simulink model "cable_driven_parallel_robot"  (R2023a)
settings: Solver=ode3  StartTime=0.0  StopTime=100  FixedStep=0.01  RelTol=1e-3
values from neighbouring files (symbols this model uses):
  cable_length = 1.2    [Model_Info.m]
  g = 9.81    [Model_Info.m]
  MP_H = 2    [Model_Info.m]
  MP_init_X = 0    [Model_Info.m]
  MP_init_Y = 0    [Model_Info.m]
  MP_init_Z = cable_length + (MP_H/2)    (= 2.2)    [Model_Info.m]
  MP_Ix = (MP_m/12)*(MP_W^2+MP_H^2)    (= 6.66666666667e-05)    [Model_Info.m]
  MP_Iy = (MP_m/12)*(MP_L^2+MP_H^2)    (= 6.66666666667e-05)    [Model_Info.m]
  MP_Iz = (MP_m/12)*(MP_L^2+MP_W^2)    (= 6.66666666667e-05)    [Model_Info.m]
  MP_L = 2    [Model_Info.m]
  MP_m = 0.0001    [Model_Info.m]
  MP_W = 2    [Model_Info.m]
  MR_init_X_L1 = -(MP_L/2)    (= -1)    [Model_Info.m]
  MR_init_X_L2 = (MP_L/2)    (= 1)    [Model_Info.m]
  MR_init_X_L3 = (MP_L/2)    (= 1)    [Model_Info.m]
  MR_init_X_L4 = -(MP_L/2)    (= -1)    [Model_Info.m]
  MR_init_Y_L1 = -(MP_W/2)    (= -1)    [Model_Info.m]
  MR_init_Y_L2 = -(MP_W/2)    (= -1)    [Model_Info.m]
  MR_init_Y_L3 = (MP_W/2)    (= 1)    [Model_Info.m]
  MR_init_Y_L4 = (MP_W/2)    (= 1)    [Model_Info.m]
  MR_init_Yaw_L1 = pi    (= 3.14159265359)    [Model_Info.m]
  MR_init_Yaw_L2 = 0    [Model_Info.m]
  MR_init_Yaw_L3 = 0    [Model_Info.m]
  MR_init_Yaw_L4 = pi    (= 3.14159265359)    [Model_Info.m]
  MR_Jr = (MR_m/12)*(MR_L^2+MR_W^2)    (= 0.333333333333)    [Model_Info.m]
  MR_m = 0.5    [Model_Info.m]
  MR_r = 2    [Model_Info.m]
  MR_WT = 2    [Model_Info.m]
  QR_Ax = 0.25*0    (= 0)    [Model_Info.m]
  QR_Ay = 0.25*0    (= 0)    [Model_Info.m]
  QR_Az = 0.25*0    (= 0)    [Model_Info.m]
  QR_b = 1.14*1e-7    (= 1.14e-07)    [Model_Info.m]
  QR_Ixx = 4.856*1e-3    (= 0.004856)    [Model_Info.m]
  QR_Iyy = 4.856*1e-3    (= 0.004856)    [Model_Info.m]
  QR_Izz = 8.801*1e-3    (= 0.008801)    [Model_Info.m]
  QR_K = 2.980*1e-6    (= 2.98e-06)    [Model_Info.m]
  QR_l = 0.225    [Model_Info.m]
  QR_m = 0.468    [Model_Info.m]
  QR_x0_U1 = -(MP_L/2)    (= -1)    [Model_Info.m]
  QR_x0_U2 = (MP_L/2)    (= 1)    [Model_Info.m]
  QR_x0_U3 = (MP_L/2)    (= 1)    [Model_Info.m]
  QR_x0_U4 = -(MP_L/2)    (= -1)    [Model_Info.m]
  QR_y0_U1 = -(MP_W/2)    (= -1)    [Model_Info.m]
  QR_y0_U2 = -(MP_W/2)    (= -1)    [Model_Info.m]
  QR_y0_U3 = (MP_W/2)    (= 1)    [Model_Info.m]
  QR_y0_U4 = (MP_W/2)    (= 1)    [Model_Info.m]
  QR_z0_U1 = 2*cable_length+(MP_H)    (= 4.4)    [Model_Info.m]
  QR_z0_U2 = 2*cable_length+(MP_H)    (= 4.4)    [Model_Info.m]
  QR_z0_U3 = 2*cable_length+(MP_H)    (= 4.4)    [Model_Info.m]
  QR_z0_U4 = 2*cable_length+(MP_H)    (= 4.4)    [Model_Info.m]
(part 1 of 12)
settings Model: Creator=ahmed  LastModifiedBy=Siddharth U
settings SolverCC: AlgebraicLoopSolver=TrustRegion
settings DebuggingCC: UnconnectedInputMsg=warning  UnconnectedOutputMsg=warning  UnconnectedLineMsg=warning  UnderSpecifiedDimensionMsg=warning
settings ModelReferenceCC: EnableRefExpFcnMdlSchedulingChecks=on

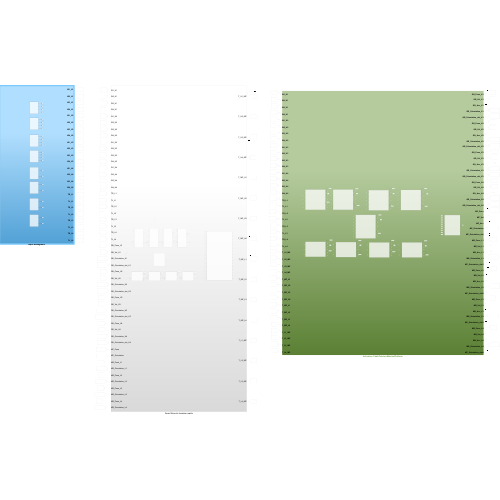
[thumbnail: Simulink's stored preview of the top-level diagram]
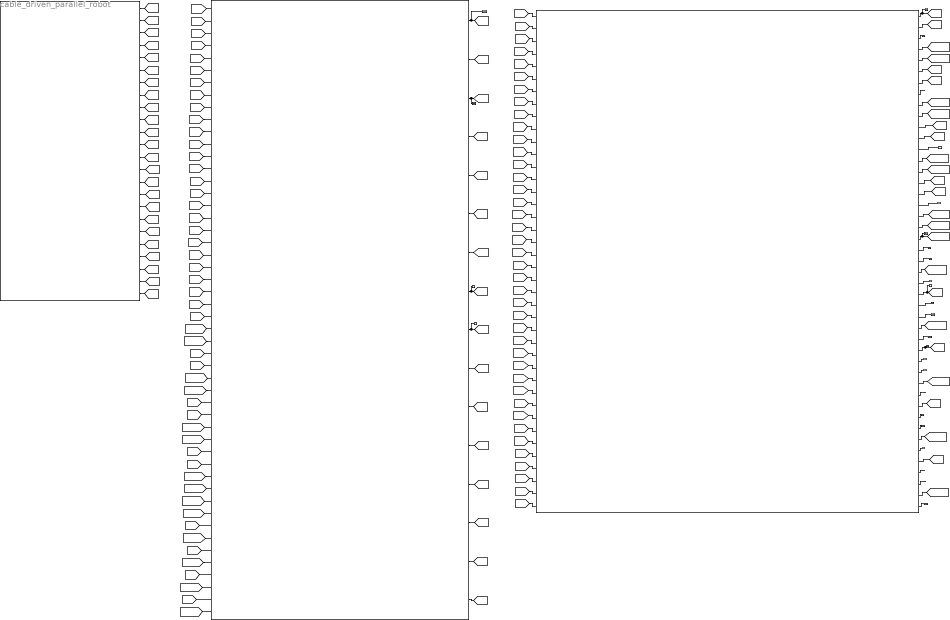
== system cable_driven_parallel_robot ==
  Actuators-CableTension-MovingPlatform : Subsystem
  Display{,1..26} (27 alike) : Display
  Input Managment : Subsystem
  Target Wrench-Jacobian matrix : Subsystem
  wires:
  Input Managment/1(W1_U1) -> [W1_U1]
  Input Managment/2(W2_U1) -> [W2_U1]
  Input Managment/3(W3_U1) -> [W3_U1]
  Input Managment/4(W4_U1) -> [W4_U1]
  Input Managment/5(W1_U2) -> [W1_U2]
  Input Managment/6(W2_U2) -> [W2_U2]
  Input Managment/7(W3_U2) -> [W3_U2]
  Input Managment/8(W4_U2) -> [W4_U2]
  Input Managment/9(W1_U3) -> [W1_U3]
  Input Managment/10(W2_U3) -> [W2_U3]
  Input Managment/11(W3_U3) -> [W3_U3]
  Input Managment/12(W4_U3) -> [W4_U3]
  Input Managment/13(W1_U4) -> [W1_U4]
  Input Managment/14(W2_U4) -> [W2_U4]
  Input Managment/15(W3_U4) -> [W3_U4]
  Input Managment/16(W4_U4) -> [W4_U4]
  Input Managment/18(TL_L1) -> [TL_L1]
  Input Managment/17(TR_L1) -> [TR_L1]
  Input Managment/20(TL_L2) -> [TL_L2]
  Input Managment/19(TR_L2) -> [TR_L2]
  Input Managment/22(TL_L3) -> [TL_L3]
  Input Managment/21(TR_L3) -> [TR_L3]
  Input Managment/24(TL_L4) -> [TL_L4]
  Input Managment/23(TR_L4) -> [TR_L4]
  [W1_U1] -> Target Wrench-Jacobian matrix/1(W1_U1)
  [W2_U1] -> Target Wrench-Jacobian matrix/2(W2_U1)
  [W3_U1] -> Target Wrench-Jacobian matrix/3(W3_U1)
  [W4_U1] -> Target Wrench-Jacobian matrix/4(W4_U1)
  [W1_U2] -> Target Wrench-Jacobian matrix/5(W1_U2)
  [W2_U2] -> Target Wrench-Jacobian matrix/6(W2_U2)
  [W3_U2] -> Target Wrench-Jacobian matrix/7(W3_U2)
  [W4_U2] -> Target Wrench-Jacobian matrix/8(W4_U2)
  [W1_U3] -> Target Wrench-Jacobian matrix/9(W1_U3)
  [W2_U3] -> Target Wrench-Jacobian matrix/10(W2_U3)
  [W3_U3] -> Target Wrench-Jacobian matrix/11(W3_U3)
  [W4_U3] -> Target Wrench-Jacobian matrix/12(W4_U3)
  [W1_U4] -> Target Wrench-Jacobian matrix/13(W1_U4)
  [W2_U4] -> Target Wrench-Jacobian matrix/14(W2_U4)
  [W3_U4] -> Target Wrench-Jacobian matrix/15(W3_U4)
  [W4_U4] -> Target Wrench-Jacobian matrix/16(W4_U4)
  [TR_L1] -> Target Wrench-Jacobian matrix/17(TR_L1)
  [TL_L1] -> Target Wrench-Jacobian matrix/18(TL_L1)
  [TR_L2] -> Target Wrench-Jacobian matrix/19(TR_L2)
  [TL_L2] -> Target Wrench-Jacobian matrix/20(TL_L2)
  [TR_L3] -> Target Wrench-Jacobian matrix/21(TR_L3)
  [TL_L3] -> Target Wrench-Jacobian matrix/22(TL_L3)
  [TR_L4] -> Target Wrench-Jacobian matrix/23(TR_L4)
  [TL_L4] -> Target Wrench-Jacobian matrix/24(TL_L4)
  [TL_L4] -> Actuators-CableTension-MovingPlatform/24(TL_L4)
  [W1_U4] -> Actuators-CableTension-MovingPlatform/13(W1_U4)
  [W4_U1] -> Actuators-CableTension-MovingPlatform/4(W4_U1)
  [TL_L1] -> Actuators-CableTension-MovingPlatform/18(TL_L1)
  [TL_L2] -> Actuators-CableTension-MovingPlatform/20(TL_L2)
  [TR_L3] -> Actuators-CableTension-MovingPlatform/21(TR_L3)
  [W3_U3] -> Actuators-CableTension-MovingPlatform/11(W3_U3)
  [TR_L1] -> Actuators-CableTension-MovingPlatform/17(TR_L1)
  [TL_L3] -> Actuators-CableTension-MovingPlatform/22(TL_L3)
  [TR_L2] -> Actuators-CableTension-MovingPlatform/19(TR_L2)
  [W4_U4] -> Actuators-CableTension-MovingPlatform/16(W4_U4)
  [TR_L4] -> Actuators-CableTension-MovingPlatform/23(TR_L4)
  [W1_U3] -> Actuators-CableTension-MovingPlatform/9(W1_U3)
  [W1_U2] -> Actuators-CableTension-MovingPlatform/5(W1_U2)
  [W3_U2] -> Actuators-CableTension-MovingPlatform/7(W3_U2)
  [W2_U3] -> Actuators-CableTension-MovingPlatform/10(W2_U3)
  [W4_U2] -> Actuators-CableTension-MovingPlatform/8(W4_U2)
  [W2_U1] -> Actuators-CableTension-MovingPlatform/2(W2_U1)
  [W2_U4] -> Actuators-CableTension-MovingPlatform/14(W2_U4)
  [W3_U1] -> Actuators-CableTension-MovingPlatform/3(W3_U1)
  [W2_U2] -> Actuators-CableTension-MovingPlatform/6(W2_U2)
  [W1_U1] -> Actuators-CableTension-MovingPlatform/1(W1_U1)
  [W4_U3] -> Actuators-CableTension-MovingPlatform/12(W4_U3)
  [W3_U4] -> Actuators-CableTension-MovingPlatform/15(W3_U4)
  Target Wrench-Jacobian matrix/1(T_U1_MP) -> Display24/1, [T_U1_MP]
  Target Wrench-Jacobian matrix/2(T_U2_MP) -> [T_U2_MP]
  Target Wrench-Jacobian matrix/3(T_U3_MP) -> Display19/1, [T_U3_MP]
  Target Wrench-Jacobian matrix/4(T_U4_MP) -> [T_U4_MP]
  Target Wrench-Jacobian matrix/6(T_MP_U2) -> [T_MP_U2]
  Target Wrench-Jacobian matrix/5(T_MP_U1) -> [T_MP_U1]
  Target Wrench-Jacobian matrix/7(T_MP_U3) -> [T_MP_U3]
  Target Wrench-Jacobian matrix/9(T_MP_L1) -> Display26/1, [T_MP_L1]
  Target Wrench-Jacobian matrix/10(T_MP_L2) -> [T_MP_L2]
  Target Wrench-Jacobian matrix/11(T_MP_L3) -> [T_MP_L3]
  Target Wrench-Jacobian matrix/12(T_MP_L4) -> [T_MP_L4]
  Target Wrench-Jacobian matrix/13(T_L1_MP) -> [T_L1_MP]
  Target Wrench-Jacobian matrix/14(T_L2_MP) -> [T_L2_MP]
  Target Wrench-Jacobian matrix/15(T_L3_MP) -> [T_L3_MP]
  Target Wrench-Jacobian matrix/16(T_L4_MP) -> [T_L4_MP]
  [T_U1_MP] -> Actuators-CableTension-MovingPlatform/25(T_U1_MP)
  [T_U3_MP] -> Actuators-CableTension-MovingPlatform/27(T_U3_MP)
  [T_U4_MP] -> Actuators-CableTension-MovingPlatform/28(T_U4_MP)
  [T_MP_U1] -> Actuators-CableTension-MovingPlatform/29(T_MP_U1)
  [T_MP_U2] -> Actuators-CableTension-MovingPlatform/30(T_MP_U2)
  [T_MP_U3] -> Actuators-CableTension-MovingPlatform/31(T_MP_U3)
  [T_MP_U4] -> Actuators-CableTension-MovingPlatform/32(T_MP_U4)
  [T_MP_L1] -> Actuators-CableTension-MovingPlatform/33(T_MP_L1)
  [T_MP_L2] -> Actuators-CableTension-MovingPlatform/34(T_MP_L2)
  [T_MP_L3] -> Actuators-CableTension-MovingPlatform/35(T_MP_L3)
  [T_MP_L4] -> Actuators-CableTension-MovingPlatform/36(T_MP_L4)
  [T_L1_MP] -> Actuators-CableTension-MovingPlatform/37(T_L1_MP)
  [T_L2_MP] -> Actuators-CableTension-MovingPlatform/38(T_L2_MP)
  [T_L3_MP] -> Actuators-CableTension-MovingPlatform/39(T_L3_MP)
  [T_L4_MP] -> Actuators-CableTension-MovingPlatform/40(T_L4_MP)
  Actuators-CableTension-MovingPlatform/1(QR_Pose_U1) -> Display23/1, [QR_Pose_U1]
  Actuators-CableTension-MovingPlatform/2(QR_Vel_U1) -> [QR_Vel_U1]
  Actuators-CableTension-MovingPlatform/4(QR_Orientation_U1) -> [QR_Orientation_U1]
  Actuators-CableTension-MovingPlatform/5(QR_Orientation_dot_U1) -> [QR_Orientation_dot_U1]
  Actuators-CableTension-MovingPlatform/6(QR_Pose_U2) -> [QR_Pose_U2]
  Actuators-CableTension-MovingPlatform/10(QR_Orientation_dot_U2) -> [QR_Orientation_dot_U2]
  Actuators-CableTension-MovingPlatform/9(QR_Orientation_U2) -> [QR_Orientation_U2]
  Actuators-CableTension-MovingPlatform/7(QR_Vel_U2) -> [QR_Vel_U2]
  Actuators-CableTension-MovingPlatform/11(QR_Pose_U3) -> [QR_Pose_U3]
  Actuators-CableTension-MovingPlatform/15(QR_Orientation_dot_U3) -> [QR_Orientation_dot_U3]
  Actuators-CableTension-MovingPlatform/14(QR_Orientation_U3) -> [QR_Orientation_U3]
  Actuators-CableTension-MovingPlatform/12(QR_Vel_U3) -> [QR_Vel_U3]
  Actuators-CableTension-MovingPlatform/16(QR_Pose_U4) -> [QR_Pose_U4]
  Actuators-CableTension-MovingPlatform/20(QR_Orientation_dot_U4) -> [QR_Orientation_dot_U4]
  Actuators-CableTension-MovingPlatform/19(QR_Orientation_U4) -> [QR_Orientation_U4]
  Actuators-CableTension-MovingPlatform/17(QR_Vel_U4) -> [QR_Vel_U4]
  Actuators-CableTension-MovingPlatform/21(MP_Pose) -> Display22/1, [MP_Pose]
  Actuators-CableTension-MovingPlatform/24(MP_Orientation) -> [MP_Orientation]
  Actuators-CableTension-MovingPlatform/26(MR_Pose_L1) -> [MR_Pose_L1], Display20/1
  Actuators-CableTension-MovingPlatform/29(MR_Orientation_L1) -> [MR_Orientation_L1]
  Actuators-CableTension-MovingPlatform/34(MR_Orientation_L2) -> [MR_Orientation_L2]
  Actuators-CableTension-MovingPlatform/39(MR_Orientation_L3) -> [MR_Orientation_L3]
  Actuators-CableTension-MovingPlatform/36(MR_Pose_L3) -> [MR_Pose_L3]
  Actuators-CableTension-MovingPlatform/44(MR_Orientation_L4) -> [MR_Orientation_L4]
  Actuators-CableTension-MovingPlatform/41(MR_Pose_L4) -> [MR_Pose_L4]
  [QR_Pose_U1] -> Target Wrench-Jacobian matrix/25(QR_Pose_U1)
  [QR_Vel_U1] -> Target Wrench-Jacobian matrix/26(QR_Vel_U1)
  [QR_Orientation_U1] -> Target Wrench-Jacobian matrix/27(QR_Orientation_U1)
  [QR_Orientation_dot_U1] -> Target Wrench-Jacobian matrix/28(QR_Orientation_dot_U1)
  [QR_Pose_U2] -> Target Wrench-Jacobian matrix/29(QR_Pose_U2)
  [QR_Vel_U2] -> Target Wrench-Jacobian matrix/30(QR_Vel_U2)
  [QR_Orientation_U2] -> Target Wrench-Jacobian matrix/31(QR_Orientation_U2)
  [QR_Orientation_dot_U2] -> Target Wrench-Jacobian matrix/32(QR_Orientation_dot_U2)
  [QR_Pose_U3] -> Target Wrench-Jacobian matrix/33(QR_Pose_U3)
  [QR_Vel_U3] -> Target Wrench-Jacobian matrix/34(QR_Vel_U3)
  [QR_Orientation_U3] -> Target Wrench-Jacobian matrix/35(QR_Orientation_U3)
  [QR_Orientation_dot_U3] -> Target Wrench-Jacobian matrix/36(QR_Orientation_dot_U3)
  [QR_Pose_U4] -> Target Wrench-Jacobian matrix/37(QR_Pose_U4)
  [QR_Vel_U4] -> Target Wrench-Jacobian matrix/38(QR_Vel_U4)
  [QR_Orientation_U4] -> Target Wrench-Jacobian matrix/39(QR_Orientation_U4)
  [QR_Orientation_dot_U4] -> Target Wrench-Jacobian matrix/40(QR_Orientation_dot_U4)
  [MP_Orientation] -> Target Wrench-Jacobian matrix/42(MP_Orientation)
  [MR_Pose_L1] -> Target Wrench-Jacobian matrix/43(MR_Pose_L1)
  [MR_Orientation_L1] -> Target Wrench-Jacobian matrix/44(MR_Orientation_L1)
  [MR_Pose_L2] -> Target Wrench-Jacobian matrix/45(MR_Pose_L2)
  [MR_Orientation_L2] -> Target Wrench-Jacobian matrix/46(MR_Orientation_L2)
  [MR_Pose_L3] -> Target Wrench-Jacobian matrix/47(MR_Pose_L3)
  [MR_Orientation_L3] -> Target Wrench-Jacobian matrix/48(MR_Orientation_L3)
  [MR_Pose_L4] -> Target Wrench-Jacobian matrix/49(MR_Pose_L4)
  [MR_Orientation_L4] -> Target Wrench-Jacobian matrix/50(MR_Orientation_L4)
  [T_U2_MP] -> Actuators-CableTension-MovingPlatform/26(T_U2_MP)
  Actuators-CableTension-MovingPlatform/3(QR_Acc_U1) -> Display/1
  Actuators-CableTension-MovingPlatform/8(QR_Acc_U2) -> Display1/1
  Actuators-CableTension-MovingPlatform/13(QR_Acc_U3) -> Display2/1
  Actuators-CableTension-MovingPlatform/18(QR_Acc_U4) -> Display3/1
  Actuators-CableTension-MovingPlatform/22(MP_Vel) -> Display4/1
  Actuators-CableTension-MovingPlatform/23(MP_Acc) -> Display5/1
  Actuators-CableTension-MovingPlatform/25(MP_Orientation_dot) -> Display6/1
  Actuators-CableTension-MovingPlatform/27(MR_Vel_L1) -> Display7/1
  Actuators-CableTension-MovingPlatform/28(MR_Acc_L1) -> Display8/1
  Actuators-CableTension-MovingPlatform/30(MP_Orientation_dot1) -> Display9/1
  Actuators-CableTension-MovingPlatform/32(MR_Vel_L2) -> Display10/1
  Actuators-CableTension-MovingPlatform/33(MR_Acc_L2) -> Display11/1
  Actuators-CableTension-MovingPlatform/35(MP_Orientation_dot2) -> Display12/1
  Actuators-CableTension-MovingPlatform/37(MR_Vel_L3) -> Display13/1
  Actuators-CableTension-MovingPlatform/38(MR_Acc_L3) -> Display14/1
  Actuators-CableTension-MovingPlatform/40(MP_Orientation_dot3) -> Display15/1
  Actuators-CableTension-MovingPlatform/42(MR_Vel_L4) -> Display16/1
  Actuators-CableTension-MovingPlatform/43(MR_Acc_L4) -> Display17/1
  Actuators-CableTension-MovingPlatform/45(MP_Orientation_dot4) -> Display18/1
  [MP_Pose] -> Target Wrench-Jacobian matrix/41(MP_Pose)
  Target Wrench-Jacobian matrix/8(T_MP_U4) -> Display25/1, [T_MP_U4]
  Actuators-CableTension-MovingPlatform/31(MR_Pose_L2) -> Display21/1, [MR_Pose_L2]

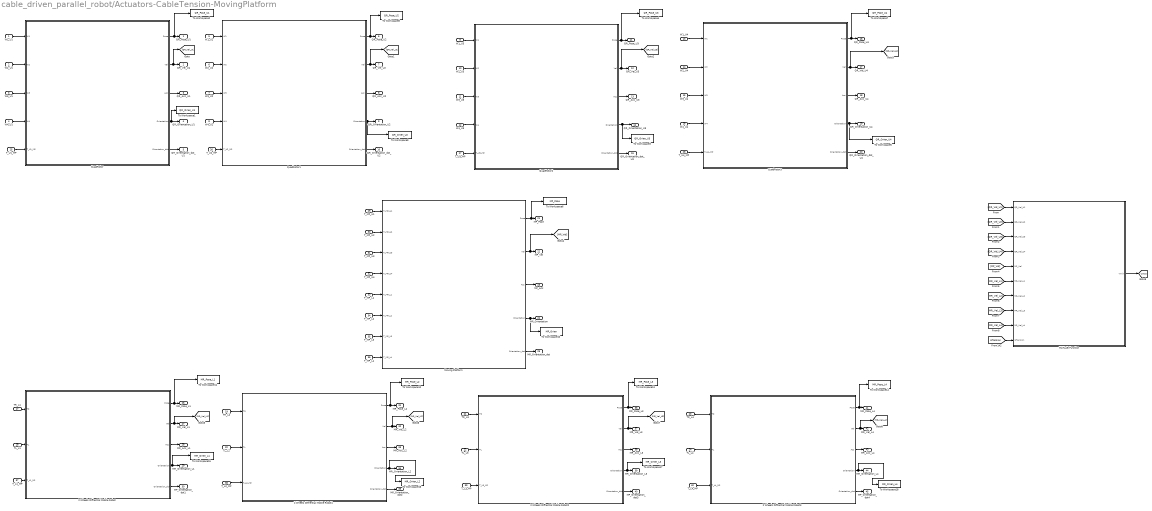
== system cable_driven_parallel_robot/Actuators-CableTension-MovingPlatform ==
  W1_U1 : Inport
  W2_U1 : Inport  Port=2
  W3_U1 : Inport  Port=3
  W4_U1 : Inport  Port=4
  W1_U2 : Inport  Port=5
  W2_U2 : Inport  Port=6
  W3_U2 : Inport  Port=7
  W4_U2 : Inport  Port=8
  W1_U3 : Inport  Port=9
  W2_U3 : Inport  Port=10
  W3_U3 : Inport  Port=11
  W4_U3 : Inport  Port=12
  W1_U4 : Inport  Port=13
  W2_U4 : Inport  Port=14
  W3_U4 : Inport  Port=15
  W4_U4 : Inport  Port=16
  TR_L1 : Inport  Port=17
  TL_L1 : Inport  Port=18
  TR_L2 : Inport  Port=19
  TL_L2 : Inport  Port=20
  TR_L3 : Inport  Port=21
  TL_L3 : Inport  Port=22
  TR_L4 : Inport  Port=23
  TL_L4 : Inport  Port=24
  T_U1_MP : Inport  Port=25
  T_U2_MP : Inport  Port=26
  T_U3_MP : Inport  Port=27
  T_U4_MP : Inport  Port=28
  T_MP_U1 : Inport  Port=29
  T_MP_U2 : Inport  Port=30
  T_MP_U3 : Inport  Port=31
  T_MP_U4 : Inport  Port=32
  T_MP_L1 : Inport  Port=33
  T_MP_L2 : Inport  Port=34
  T_MP_L3 : Inport  Port=35
  T_MP_L4 : Inport  Port=36
  T_L1_MP : Inport  Port=37
  T_L2_MP : Inport  Port=38
  T_L3_MP : Inport  Port=39
  T_L4_MP : Inport  Port=40
  2 Wheels Diffrential Mobile Robot : Subsystem
  2 Wheels Diffrential Mobile Robot1 : Subsystem
  2 Wheels Diffrential Mobile Robot2 : Subsystem
  2 Wheels Diffrential Mobile Robot3 : Subsystem
  MATLAB Function : MATLAB Function  TreatAsAtomicUnit=on
  Moving Platform : Subsystem
  QuadRotor : Subsystem
  QuadRotor1 : Subsystem
  QuadRotor2 : Subsystem
  QuadRotor3 : Subsystem
  To Workspace1 : ToWorkspace  VariableName=QR_Orien_U1  SampleTime=-1
      settings: Save2DSignal=2-D array (concatenate along first dimension)
  To Workspace10 : ToWorkspace  VariableName=MP_Orien  SampleTime=-1
      settings: Save2DSignal=2-D array (concatenate along first dimension)
  To Workspace11 : ToWorkspace  VariableName=MR_Pose_L1  SampleTime=-1
      settings: Save2DSignal=2-D array (concatenate along first dimension)
  To Workspace12 : ToWorkspace  VariableName=MR_Pose_L2  SampleTime=-1
      settings: Save2DSignal=2-D array (concatenate along first dimension)
  To Workspace13 : ToWorkspace  VariableName=MR_Pose_L3  SampleTime=-1
      settings: Save2DSignal=2-D array (concatenate along first dimension)
  To Workspace14 : ToWorkspace  VariableName=MR_Pose_L4  SampleTime=-1
      settings: Save2DSignal=2-D array (concatenate along first dimension)
  To Workspace15 : ToWorkspace  VariableName=MR_Orien_L1  SampleTime=-1
      settings: Save2DSignal=2-D array (concatenate along first dimension)
  To Workspace16 : ToWorkspace  VariableName=MR_Orien_L2  SampleTime=-1
      settings: Save2DSignal=2-D array (concatenate along first dimension)
  To Workspace17 : ToWorkspace  VariableName=MR_Orien_L3  SampleTime=-1
      settings: Save2DSignal=2-D array (concatenate along first dimension)
  To Workspace18 : ToWorkspace  VariableName=MR_Orien_L4  SampleTime=-1
      settings: Save2DSignal=2-D array (concatenate along first dimension)
  To Workspace2 : ToWorkspace  VariableName=QR_Pose_U1  SampleTime=-1
      settings: Save2DSignal=2-D array (concatenate along first dimension)
  To Workspace3 : ToWorkspace  VariableName=QR_Orien_U3  SampleTime=-1
      settings: Save2DSignal=2-D array (concatenate along first dimension)
  To Workspace4 : ToWorkspace  VariableName=QR_Pose_U3  SampleTime=-1
      settings: Save2DSignal=2-D array (concatenate along first dimension)
  To Workspace5 : ToWorkspace  VariableName=QR_Orien_U4  SampleTime=-1
      settings: Save2DSignal=2-D array (concatenate along first dimension)
  To Workspace6 : ToWorkspace  VariableName=MP_Pose  SampleTime=-1
      settings: Save2DSignal=2-D array (concatenate along first dimension)
  To Workspace7 : ToWorkspace  VariableName=QR_Pose_U4  SampleTime=-1
      settings: Save2DSignal=2-D array (concatenate along first dimension)
  To Workspace8 : ToWorkspace  VariableName=QR_Pose_U2  SampleTime=-1
      settings: Save2DSignal=2-D array (concatenate along first dimension)
  To Workspace9 : ToWorkspace  VariableName=QR_Orien_U2  SampleTime=-1
      settings: Save2DSignal=2-D array (concatenate along first dimension)
  QR_Pose_U1 : Outport
  QR_Vel_U1 : Outport  Port=2
  QR_Acc_U1 : Outport  Port=3
  QR_Orientation_U1 : Outport  Port=4
  QR_Orientation_dot_U1 : Outport  Port=5
  QR_Pose_U2 : Outport  Port=6
  QR_Vel_U2 : Outport  Port=7
  QR_Acc_U2 : Outport  Port=8
  QR_Orientation_U2 : Outport  Port=9
  QR_Orientation_dot_U2 : Outport  Port=10
  QR_Pose_U3 : Outport  Port=11
  QR_Vel_U3 : Outport  Port=12
  QR_Acc_U3 : Outport  Port=13
  QR_Orientation_U3 : Outport  Port=14
  QR_Orientation_dot_U3 : Outport  Port=15
  QR_Pose_U4 : Outport  Port=16
  QR_Vel_U4 : Outport  Port=17
  QR_Acc_U4 : Outport  Port=18
  QR_Orientation_U4 : Outport  Port=19
  QR_Orientation_dot_U4 : Outport  Port=20
  MP_Pose : Outport  Port=21
  MP_Vel : Outport  Port=22
  MP_Acc : Outport  Port=23
  MP_Orientation : Outport  Port=24
  MP_Orientation_dot : Outport  Port=25
  MR_Pose_L1 : Outport  Port=26
  MR_Vel_L1 : Outport  Port=27
  MR_Acc_L1 : Outport  Port=28
  MR_Orientation_L1 : Outport  Port=29
  MP_Orientation_dot1 : Outport  Port=30
  MR_Pose_L2 : Outport  Port=31
  MR_Vel_L2 : Outport  Port=32
  MR_Acc_L2 : Outport  Port=33
  MR_Orientation_L2 : Outport  Port=34
  MP_Orientation_dot2 : Outport  Port=35
  MR_Pose_L3 : Outport  Port=36
  MR_Vel_L3 : Outport  Port=37
  MR_Acc_L3 : Outport  Port=38
  MR_Orientation_L3 : Outport  Port=39
  MP_Orientation_dot3 : Outport  Port=40
  MR_Pose_L4 : Outport  Port=41
  MR_Vel_L4 : Outport  Port=42
  MR_Acc_L4 : Outport  Port=43
  MR_Orientation_L4 : Outport  Port=44
  MP_Orientation_dot4 : Outport  Port=45
  tag scope: Vmin=global
  wires:
  W3_U1/1 -> QuadRotor/3(W3)
  W1_U2/1 -> QuadRotor1/1(W1)
  QuadRotor/1(Pose) -> To Workspace2/1, QR_Pose_U1/1
  W2_U1/1 -> QuadRotor/2(W2)
  T_L2_MP/1 -> 2 Wheels Diffrential Mobile Robot1/3(T_L2_MP)
  W1_U4/1 -> QuadRotor3/1(W1)
  W4_U4/1 -> QuadRotor3/4(W4)
  W1_U1/1 -> QuadRotor/1(W1)
  W3_U4/1 -> QuadRotor3/3(W3)
  W4_U1/1 -> QuadRotor/4(W4)
  W3_U2/1 -> QuadRotor1/3(W3)
  T_L3_MP/1 -> 2 Wheels Diffrential Mobile Robot2/3(T_L3_MP)
  T_L4_MP/1 -> 2 Wheels Diffrential Mobile Robot3/3(T_L4_MP)
  QuadRotor/4(Orientation) -> To Workspace1/1, QR_Orientation_U1/1
  QuadRotor/3(Acc) -> QR_Acc_U1/1
  TR_L1/1 -> 2 Wheels Diffrential Mobile Robot/1(TR)
  TR_L4/1 -> 2 Wheels Diffrential Mobile Robot3/1(TR)
  QuadRotor/2(Vel) -> [QR_Vel_U1], QR_Vel_U1/1
  W2_U2/1 -> QuadRotor1/2(W2)
  T_L1_MP/1 -> 2 Wheels Diffrential Mobile Robot/3(T_L1_MP)
  TL_L1/1 -> 2 Wheels Diffrential Mobile Robot/2(TL)
  W4_U2/1 -> QuadRotor1/4(W4)
  QuadRotor/5(Orientation_dot) -> QR_Orientation_dot_U1/1
  T_U1_MP/1 -> QuadRotor/5(T_U1_MP)
  TL_L4/1 -> 2 Wheels Diffrential Mobile Robot3/2(TL)
  W2_U4/1 -> QuadRotor3/2(W2)
  T_U2_MP/1 -> QuadRotor1/5(T_U2_MP)
  T_U3_MP/1 -> QuadRotor2/5(T_U3_MP)
  T_U4_MP/1 -> QuadRotor3/5(T_U4_MP)
  T_MP_U1/1 -> Moving Platform/1(T_MP_U1)
  T_MP_U2/1 -> Moving Platform/2("T_MP_U2 ")
  T_MP_U3/1 -> Moving Platform/3(T_MP_U3)
  T_MP_U4/1 -> Moving Platform/4(T_MP_U4)
  T_MP_L1/1 -> Moving Platform/5(T_MP_L1)
  T_MP_L2/1 -> Moving Platform/6(T_MP_L2)
  T_MP_L3/1 -> Moving Platform/7(T_MP_L3)
  T_MP_L4/1 -> Moving Platform/8(T_MP_L4)
  QuadRotor1/4(Orientation) -> QR_Orientation_U2/1, To Workspace9/1
  QuadRotor1/3(Acc) -> QR_Acc_U2/1
  QuadRotor1/2(Vel) -> [QR_Vel_U2], QR_Vel_U2/1
  QuadRotor1/5(Orientation_dot) -> QR_Orientation_dot_U2/1
  QuadRotor1/1(Pose) -> To Workspace8/1, QR_Pose_U2/1
  QuadRotor2/3(Acc) -> QR_Acc_U3/1
  QuadRotor2/2(Vel) -> [QR_Vel_U3], QR_Vel_U3/1
  QuadRotor2/5(Orientation_dot) -> QR_Orientation_dot_U3/1
  QuadRotor2/1(Pose) -> To Workspace4/1, QR_Pose_U3/1
  QuadRotor3/4(Orientation) -> QR_Orientation_U4/1, To Workspace5/1
  QuadRotor3/3(Acc) -> QR_Acc_U4/1
  QuadRotor3/2(Vel) -> [QR_Vel_U4], QR_Vel_U4/1
  QuadRotor3/5(Orientation_dot) -> QR_Orientation_dot_U4/1
  QuadRotor3/1(Pose) -> To Workspace7/1, QR_Pose_U4/1
  Moving Platform/4(Orientation) -> To Workspace10/1, MP_Orientation/1
  Moving Platform/3(Acc) -> MP_Acc/1
  Moving Platform/2(Vel) -> [MP_Vel], MP_Vel/1
  Moving Platform/5(Orientation_dot) -> MP_Orientation_dot/1
  Moving Platform/1(Pose) -> To Workspace6/1, MP_Pose/1
  2 Wheels Diffrential Mobile Robot/1(Pose) -> To Workspace11/1, MR_Pose_L1/1
  2 Wheels Diffrential Mobile Robot/3(Acc) -> MR_Acc_L1/1
  2 Wheels Diffrential Mobile Robot/5(Orientation_dot) -> MP_Orientation_dot1/1
  2 Wheels Diffrential Mobile Robot/2(Vel) -> [MR_Vel_L1], MR_Vel_L1/1
  2 Wheels Diffrential Mobile Robot/4(Orientation) -> To Workspace15/1, MR_Orientation_L1/1
  2 Wheels Diffrential Mobile Robot1/5(Orientation_dot) -> MP_Orientation_dot2/1
  2 Wheels Diffrential Mobile Robot1/1(Pose) -> To Workspace12/1, MR_Pose_L2/1
  2 Wheels Diffrential Mobile Robot1/3(Acc) -> MR_Acc_L2/1
  2 Wheels Diffrential Mobile Robot1/2(Vel) -> [MR_Vel_L2], MR_Vel_L2/1
  2 Wheels Diffrential Mobile Robot1/4(Orientation) -> To Workspace16/1, MR_Orientation_L2/1
  2 Wheels Diffrential Mobile Robot2/5(Orientation_dot) -> MP_Orientation_dot3/1
  2 Wheels Diffrential Mobile Robot2/1(Pose) -> To Workspace13/1, MR_Pose_L3/1
  2 Wheels Diffrential Mobile Robot2/3(Acc) -> MR_Acc_L3/1
  2 Wheels Diffrential Mobile Robot2/2(Vel) -> [MR_Vel_L3], MR_Vel_L3/1
  2 Wheels Diffrential Mobile Robot2/4(Orientation) -> To Workspace17/1, MR_Orientation_L3/1
  2 Wheels Diffrential Mobile Robot3/5(Orientation_dot) -> MP_Orientation_dot4/1
  2 Wheels Diffrential Mobile Robot3/1(Pose) -> To Workspace14/1, MR_Pose_L4/1
  2 Wheels Diffrential Mobile Robot3/3(Acc) -> MR_Acc_L4/1
  2 Wheels Diffrential Mobile Robot3/2(Vel) -> [MR_Vel_L4], MR_Vel_L4/1
  2 Wheels Diffrential Mobile Robot3/4(Orientation) -> To Workspace18/1, MR_Orientation_L4/1
  W1_U3/1 -> QuadRotor2/1(W1)
  W4_U3/1 -> QuadRotor2/4(W4)
  W2_U3/1 -> QuadRotor2/2(W2)
  W3_U3/1 -> QuadRotor2/3(W3)
  TL_L2/1 -> 2 Wheels Diffrential Mobile Robot1/2(TL)
  TR_L2/1 -> 2 Wheels Diffrential Mobile Robot1/1(TR)
  TL_L3/1 -> 2 Wheels Diffrential Mobile Robot2/2(TL)
  TR_L3/1 -> 2 Wheels Diffrential Mobile Robot2/1(TR)
  QuadRotor2/4(Orientation) -> To Workspace3/1, QR_Orientation_U3/1
  [QR_Vel_U1] -> MATLAB Function/1(QR_Vel_U1)
  [QR_Vel_U2] -> MATLAB Function/2(QR_Vel_U2)
  [QR_Vel_U3] -> MATLAB Function/3(QR_Vel_U3)
  [QR_Vel_U4] -> MATLAB Function/4(QR_Vel_U4)
  [MP_Vel] -> MATLAB Function/5(MP_Vel)
  [MR_Vel_L1] -> MATLAB Function/6(MR_Vel_L1)
  [MR_Vel_L2] -> MATLAB Function/7(MR_Vel_L2)
  [MR_Vel_L3] -> MATLAB Function/8(MR_Vel_L3)
  [MR_Vel_L4] -> MATLAB Function/9(MR_Vel_L4)
  [isTension] -> MATLAB Function/10(isTension)
  MATLAB Function/1(Vmin) -> [Vmin]

== system cable_driven_parallel_robot/Input Managment ==
  MR_Input_L1 : Subsystem
  MR_Input_L2 : Subsystem
  MR_Input_L3 : Subsystem
  MR_Input_L4 : Subsystem
  QR_Input_U1 : Subsystem
  QR_Input_U2 : Subsystem
  QR_Input_U3 : Subsystem
  QR_Input_U4 : Subsystem
  W1_U1 : Outport
  W2_U1 : Outport  Port=2
  W3_U1 : Outport  Port=3
  W4_U1 : Outport  Port=4
  W1_U2 : Outport  Port=5
  W2_U2 : Outport  Port=6
  W3_U2 : Outport  Port=7
  W4_U2 : Outport  Port=8
  W1_U3 : Outport  Port=9
  W2_U3 : Outport  Port=10
  W3_U3 : Outport  Port=11
  W4_U3 : Outport  Port=12
  W1_U4 : Outport  Port=13
  W2_U4 : Outport  Port=14
  W3_U4 : Outport  Port=15
  W4_U4 : Outport  Port=16
  TR_L1 : Outport  Port=17
  TL_L1 : Outport  Port=18
  TR_L2 : Outport  Port=19
  TL_L2 : Outport  Port=20
  TR_L3 : Outport  Port=21
  TL_L3 : Outport  Port=22
  TR_L4 : Outport  Port=23
  TL_L4 : Outport  Port=24
  wires:
  QR_Input_U2/4(W4_U2) -> W4_U2/1
  QR_Input_U2/3(W3_U2) -> W3_U2/1
  QR_Input_U2/2(W2_U2) -> W2_U2/1
  QR_Input_U2/1(W1_U2) -> W1_U2/1
  QR_Input_U3/4(W4_U3) -> W4_U3/1
  QR_Input_U3/3(W3_U3) -> W3_U3/1
  QR_Input_U3/2(W2_U3) -> W2_U3/1
  QR_Input_U3/1(W1_U3) -> W1_U3/1
  QR_Input_U4/4(W4_U4) -> W4_U4/1
  QR_Input_U4/3(W3_U4) -> W3_U4/1
  QR_Input_U4/2(W2_U4) -> W2_U4/1
  QR_Input_U4/1(W1_U4) -> W1_U4/1
  MR_Input_L1/1(TR_L1) -> TR_L1/1
  MR_Input_L1/2(TL_L1) -> TL_L1/1
  MR_Input_L2/1(TR_L2) -> TR_L2/1
  MR_Input_L2/2(TL_L2) -> TL_L2/1
  MR_Input_L3/1(TR_L3) -> TR_L3/1
  MR_Input_L3/2(TL_L3) -> TL_L3/1
  MR_Input_L4/1(TR_L4) -> TR_L4/1
  MR_Input_L4/2(TL_L4) -> TL_L4/1

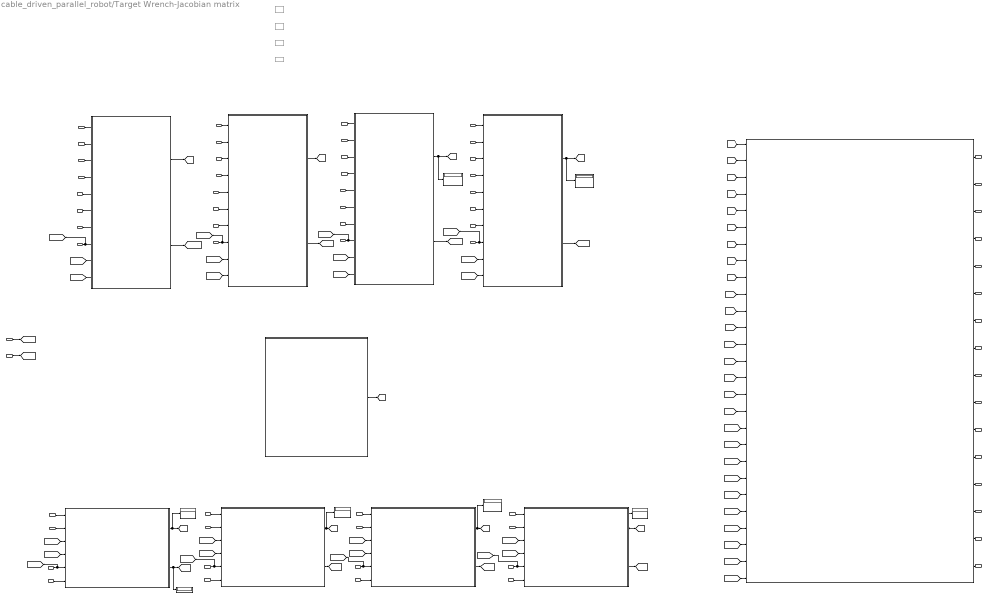
== system cable_driven_parallel_robot/Target Wrench-Jacobian matrix ==
  W1_U1 : Inport
  W2_U1 : Inport  Port=2
  W3_U1 : Inport  Port=3
  W4_U1 : Inport  Port=4
  W1_U2 : Inport  Port=5
  W2_U2 : Inport  Port=6
  W3_U2 : Inport  Port=7
  W4_U2 : Inport  Port=8
  W1_U3 : Inport  Port=9
  W2_U3 : Inport  Port=10
  W3_U3 : Inport  Port=11
  W4_U3 : Inport  Port=12
  W1_U4 : Inport  Port=13
  W2_U4 : Inport  Port=14
  W3_U4 : Inport  Port=15
  W4_U4 : Inport  Port=16
  TR_L1 : Inport  Port=17
  TL_L1 : Inport  Port=18
  TR_L2 : Inport  Port=19
  TL_L2 : Inport  Port=20
  TR_L3 : Inport  Port=21
  TL_L3 : Inport  Port=22
  TR_L4 : Inport  Port=23
  TL_L4 : Inport  Port=24
  QR_Pose_U1 : Inport  Port=25  PortDimensions=3
  QR_Vel_U1 : Inport  Port=26  PortDimensions=3
  QR_Orientation_U1 : Inport  Port=27  PortDimensions=3
  QR_Orientation_dot_U1 : Inport  Port=28  PortDimensions=3
  QR_Pose_U2 : Inport  Port=29  PortDimensions=3
  QR_Vel_U2 : Inport  Port=30  PortDimensions=3
  QR_Orientation_U2 : Inport  Port=31  PortDimensions=3
  QR_Orientation_dot_U2 : Inport  Port=32  PortDimensions=3
  QR_Pose_U3 : Inport  Port=33  PortDimensions=3
  QR_Vel_U3 : Inport  Port=34  PortDimensions=3
  QR_Orientation_U3 : Inport  Port=35  PortDimensions=3
  QR_Orientation_dot_U3 : Inport  Port=36  PortDimensions=3
  QR_Pose_U4 : Inport  Port=37  PortDimensions=3
  QR_Vel_U4 : Inport  Port=38  PortDimensions=3
  QR_Orientation_U4 : Inport  Port=39  PortDimensions=3
  QR_Orientation_dot_U4 : Inport  Port=40  PortDimensions=3
  MP_Pose : Inport  Port=41  PortDimensions=3
  MP_Orientation : Inport  Port=42  PortDimensions=3
  MR_Pose_L1 : Inport  Port=43  PortDimensions=3
  MR_Orientation_L1 : Inport  Port=44  PortDimensions=3
  MR_Pose_L2 : Inport  Port=45  PortDimensions=3
  MR_Orientation_L2 : Inport  Port=46  PortDimensions=3
  MR_Pose_L3 : Inport  Port=47  PortDimensions=3
  MR_Orientation_L3 : Inport  Port=48  PortDimensions=3
  MR_Pose_L4 : Inport  Port=49  PortDimensions=3
  MR_Orientation_L4 : Inport  Port=50  PortDimensions=3
  2 Wheels Diffrential Mobile Robot L1 : Subsystem
  2 Wheels Diffrential Mobile Robot L2 : Subsystem
  2 Wheels Diffrential Mobile Robot L3 : Subsystem
  2 Wheels Diffrential Mobile Robot L4 : Subsystem
  Display{,1..6} (7 alike) : Display
  Moving Platform : Subsystem
  Omega 17 : Constant  Commented=on  Value=638.2990
  Omega 18 : Constant  Commented=on  Value=607.1625
  Omega 19 : Constant  Commented=on  Value=638.2990
  Omega 20 : Constant  Commented=on  Value=607.1625
  QuadRotor U1 : Subsystem
  QuadRotor U2 : Subsystem
  QuadRotor U3 : Subsystem
  QuadRotor U4 : Subsystem
  Subsystem : Subsystem
  T_U1_MP : Outport
  T_U2_MP : Outport  Port=2
  T_U3_MP : Outport  Port=3
  T_U4_MP : Outport  Port=4
  T_MP_U1 : Outport  Port=5
  T_MP_U2 : Outport  Port=6
  T_MP_U3 : Outport  Port=7
  T_MP_U4 : Outport  Port=8
  T_MP_L1 : Outport  Port=9
  T_MP_L2 : Outport  Port=10
  T_MP_L3 : Outport  Port=11
  T_MP_L4 : Outport  Port=12
  T_L1_MP : Outport  Port=13
  T_L2_MP : Outport  Port=14
  T_L3_MP : Outport  Port=15
  T_L4_MP : Outport  Port=16
  wires:
  2 Wheels Diffrential Mobile Robot L4/2("isTension_L4 ") -> [isTension_L4]
  [QR_F_U3] -> Subsystem/3(QR_F_U3)
  QR_Orientation_U1/1 -> QuadRotor U1/6("QR_Orientation_U1 ")
  [isTension_U3] -> Subsystem/12(isTension_U3)
  QuadRotor U4/2(isTension_U4) -> [isTension_U4]
  [QR_F_U4] -> Subsystem/4(QR_F_U4)
  QuadRotor U4/1(QR_F_U4) -> Display/1, [QR_F_U4]
  [isTension_L4] -> Subsystem/17(isTension_L4)
  [QR_F_U2] -> Subsystem/2(QR_F_U2)
  2 Wheels Diffrential Mobile Robot L2/1(MR_F_L2) -> Display1/1, [MR_F_L2]
  [isTension_U1] -> Subsystem/10(isTension_U1)
  [isTension_U4] -> Subsystem/13(isTension_U4)
  Moving Platform/1(MP_F) -> [MP_F]
  2 Wheels Diffrential Mobile Robot L3/1(MR_F_L3) -> Display2/1, [MR_F_L3]
  [MR_F_L1] -> Subsystem/6(MR_F_L1)
  [MP_F] -> Subsystem/5(MP_F)
  [QR_F_U1] -> Subsystem/1(QR_F_U1)
  QuadRotor U2/1(QR_F_U2) -> [QR_F_U2]
  [MR_F_L2] -> Subsystem/7(MR_F_L2)
  QuadRotor U1/2(isTension_U1) -> [isTension_U1]
  [isTension_L1] -> Subsystem/14(isTension_L1)
  2 Wheels Diffrential Mobile Robot L1/2("isTension_L1 ") -> Display4/1, [isTension_L1]
  [isTension_L2] -> Subsystem/15(isTension_L2)
  QuadRotor U3/1(QR_F_U3) -> Display3/1, [QR_F_U3]
  QuadRotor U3/2(isTension_U3) -> [isTension_U3]
  QuadRotor U1/1(QR_F_U1) -> [QR_F_U1]
  QuadRotor U2/2(isTension_U2) -> [isTension_U2]
  [MR_F_L3] -> Subsystem/8(MR_F_L3)
  QR_Vel_U1/1 -> QuadRotor U1/5("QR_Vel_U1 ")
  2 Wheels Diffrential Mobile Robot L4/1(MR_F_L4) -> Display5/1, [MR_F_L4]
  2 Wheels Diffrential Mobile Robot L3/2("isTension_L3 ") -> [isTension_L3]
  [isTension_L3] -> Subsystem/16(isTension_L3)
  [MR_F_L4] -> Subsystem/9(MR_F_L4)
  2 Wheels Diffrential Mobile Robot L2/2("isTension_L2 ") -> [isTension_L2]
  [isTension_U2] -> Subsystem/11(isTension_U2)
  QR_Pose_U1/1 -> [QR_Pose_U1], QuadRotor U1/8("QR_Pose_U1 ")
  Subsystem/1(T_MP_U1) -> T_MP_U1/1
  QR_Orientation_dot_U1/1 -> QuadRotor U1/7("QR_Orientation_dot_U1 ")
  MR_Pose_L1/1 -> [MR_Pose_L1], 2 Wheels Diffrential Mobile Robot L1/5("MR_Pose_L1 ")
  MR_Orientation_L1/1 -> 2 Wheels Diffrential Mobile Robot L1/6(MR_Orientation_L1)
  Subsystem/3(T_MP_U2) -> T_MP_U2/1
  Subsystem/5(T_MP_U3) -> T_MP_U3/1
  Subsystem/7(T_MP_U4) -> T_MP_U4/1
  Subsystem/9(T_MP_L1) -> T_MP_L1/1
  Subsystem/11(T_MP_L2) -> T_MP_L2/1
  Subsystem/13(T_MP_L3) -> T_MP_L3/1
  Subsystem/15(T_MP_L4) -> T_MP_L4/1
  Subsystem/2(T_U1_MP) -> T_U1_MP/1
  Subsystem/4(T_U2_MP) -> T_U2_MP/1
  Subsystem/6(T_U3_MP) -> T_U3_MP/1
  Subsystem/8(T_U4_MP) -> T_U4_MP/1
  Subsystem/10(T_L1_MP) -> T_L1_MP/1
  Subsystem/12(T_L2_MP) -> T_L2_MP/1
  Subsystem/14(T_L3_MP) -> T_L3_MP/1
  Subsystem/16(T_L4_MP) -> T_L4_MP/1
  MP_Pose/1 -> [MP_Pose]
  MP_Orientation/1 -> [MP_Orientation]
  [MP_Pose] -> QuadRotor U1/9(MP_Pose)
  [MP_Orientation] -> QuadRotor U1/10(MP_Orientation)
  QR_Orientation_dot_U2/1 -> QuadRotor U2/7("QR_Orientation_dot_U2 ")
  QR_Vel_U2/1 -> QuadRotor U2/5("QR_Vel_U2 ")
  QR_Orientation_U2/1 -> QuadRotor U2/6("QR_Orientation_U2 ")
  [MP_Orientation] -> QuadRotor U2/10(MP_Orientation)
  QR_Pose_U2/1 -> [QR_Pose_U2], QuadRotor U2/8(QR_Pose_U2)
  [MP_Pose] -> QuadRotor U2/9(MP_Pose)
  QR_Orientation_dot_U3/1 -> QuadRotor U3/7("QR_Orientation_dot_U3 ")
  QR_Vel_U3/1 -> QuadRotor U3/5("QR_Vel_U3 ")
  QR_Orientation_U3/1 -> QuadRotor U3/6("QR_Orientation_U3 ")
  [MP_Orientation] -> QuadRotor U3/10(MP_Orientation)
  QR_Pose_U3/1 -> [QR_Pose_U3], QuadRotor U3/8("QR_Pose_U3 ")
  [MP_Pose] -> QuadRotor U3/9(MP_Pose)
  QR_Orientation_dot_U4/1 -> QuadRotor U4/7("QR_Orientation_dot_U4 ")
  QR_Orientation_U4/1 -> QuadRotor U4/6("QR_Orientation_U4 ")
  QR_Pose_U4/1 -> [QR_Pose_U4], QuadRotor U4/8("QR_Pose_U4 ")
  [MP_Orientation] -> QuadRotor U4/10(MP_Orientation)
  [MP_Pose] -> QuadRotor U4/9(MP_Pose)
  QR_Vel_U4/1 -> QuadRotor U4/5("QR_Vel_U4 ")
  [MP_Orientation] -> 2 Wheels Diffrential Mobile Robot L1/4(MP_Orientation)
  [MP_Pose] -> 2 Wheels Diffrential Mobile Robot L1/3(MP_Pose)
  [MP_Pose] -> 2 Wheels Diffrential Mobile Robot L2/3(MP_Pose)
  [MP_Orientation] -> 2 Wheels Diffrential Mobile Robot L2/4(MP_Orientation)
  MR_Orientation_L2/1 -> 2 Wheels Diffrential Mobile Robot L2/6(MR_Orientation_L2)
  MR_Pose_L2/1 -> [MR_Pose_L2], 2 Wheels Diffrential Mobile Robot L2/5("MR_Pose_L2 ")
  MR_Orientation_L3/1 -> 2 Wheels Diffrential Mobile Robot L3/6(MR_Orientation_L3)
  MR_Pose_L3/1 -> [MR_Pose_L3], 2 Wheels Diffrential Mobile Robot L3/5("MR_Pose_L3 ")
  [MP_Orientation] -> 2 Wheels Diffrential Mobile Robot L3/4(MP_Orientation)
  [MP_Pose] -> 2 Wheels Diffrential Mobile Robot L3/3(MP_Pose)
  MR_Orientation_L4/1 -> 2 Wheels Diffrential Mobile Robot L4/6(MR_Orientation_L4)
  MR_Pose_L4/1 -> [MR_Pose_L4], 2 Wheels Diffrential Mobile Robot L4/5("MR_Pose_L4 ")
  [MP_Orientation] -> 2 Wheels Diffrential Mobile Robot L4/4(MR_Orientation)
  [MP_Pose] -> 2 Wheels Diffrential Mobile Robot L4/3(MP_Pose)
  W3_U1/1 -> QuadRotor U1/3(W3)
  W2_U1/1 -> QuadRotor U1/2(W2)
  W1_U1/1 -> QuadRotor U1/1(W1)
  W4_U1/1 -> QuadRotor U1/4(W4)
  W2_U2/1 -> QuadRotor U2/2(W2)
  W3_U2/1 -> QuadRotor U2/3(W3)
  W1_U2/1 -> QuadRotor U2/1(W1)
  W4_U2/1 -> QuadRotor U2/4(W4)
  W2_U3/1 -> QuadRotor U3/2(W2)
  W3_U3/1 -> QuadRotor U3/3(W3)
  W1_U3/1 -> QuadRotor U3/1(W1)
  W4_U3/1 -> QuadRotor U3/4(W4)
  W2_U4/1 -> QuadRotor U4/2(W2)
  W3_U4/1 -> QuadRotor U4/3(W3)
  W1_U4/1 -> QuadRotor U4/1(W1)
  W4_U4/1 -> QuadRotor U4/4(W4)
  TL_L1/1 -> 2 Wheels Diffrential Mobile Robot L1/2(TL_L1)
  TR_L1/1 -> 2 Wheels Diffrential Mobile Robot L1/1(TR_L1)
  TL_L2/1 -> 2 Wheels Diffrential Mobile Robot L2/2(TL_L2)
  TR_L2/1 -> 2 Wheels Diffrential Mobile Robot L2/1(TR_L2)
  TL_L3/1 -> 2 Wheels Diffrential Mobile Robot L3/2(TL_L3)
  TR_L3/1 -> 2 Wheels Diffrential Mobile Robot L3/1(TR_L3)
  TL_L4/1 -> 2 Wheels Diffrential Mobile Robot L4/2(TL_L4)
  TR_L4/1 -> 2 Wheels Diffrential Mobile Robot L4/1(TR_L4)
  [MP_Orientation] -> Subsystem/22(MP_Orientation)
  [MP_Pose] -> Subsystem/23(MP_Pose)
  [MR_Pose_L4] -> Subsystem/27(MR_Pose_L4)
  [MR_Pose_L3] -> Subsystem/26(MR_Pose_L3)
  [MR_Pose_L2] -> Subsystem/25(MR_Pose_L2)
  [MR_Pose_L1] -> Subsystem/24(MR_Pose_L1)
  [QR_Pose_U4] -> Subsystem/21(QR_Pose_U4)
  [QR_Pose_U3] -> Subsystem/20(QR_Pose_U3)
  [QR_Pose_U2] -> Subsystem/19(QR_Pose_U2)
  [QR_Pose_U1] -> Subsystem/18(QR_Pose_U1)
  2 Wheels Diffrential Mobile Robot L1/1(MR_F_L1) -> Display6/1, [MR_F_L1]

== system cable_driven_parallel_robot/Actuators-CableTension-MovingPlatform/2 Wheels Diffrential Mobile Robot ==
  TR : Inport
  TL : Inport  Port=2
  T_L1_MP : Inport  Port=3
  2 Wheels Diffrential Mobile Robot : Subsystem
  Constant{,1..5} (6 alike) : Constant  Value=0
  Constant17 : Constant  Value=MR_Jr
  Constant18 : Constant  Value=MR_m
  Constant19 : Constant  Value=MR_r
  Constant20 : Constant  Value=MR_WT
  Delay22 : Delay  DelayLength=1
  IC : InitialCondition  Value=MR_init_Yaw_L1
  MATLAB Function7 : MATLAB Function  TreatAsAtomicUnit=on
  Mux{,1..4} (5 alike) : Mux  Inputs=3
  Pose : Outport
  Vel : Outport  Port=2
  Acc : Outport  Port=3
  Orientation : Outport  Port=4
  Orientation_dot : Outport  Port=5
  wires:
  Constant19/1 -> 2 Wheels Diffrential Mobile Robot/8(r)
  Constant17/1 -> 2 Wheels Diffrential Mobile Robot/6(Jr)
  Constant18/1 -> 2 Wheels Diffrential Mobile Robot/7(mass)
  Constant20/1 -> 2 Wheels Diffrential Mobile Robot/9(Wheel Track)
  TL/1 -> 2 Wheels Diffrential Mobile Robot/2(TL)
  TR/1 -> 2 Wheels Diffrential Mobile Robot/1(TR)
  Constant/1 -> Mux1/1
  [z] -> Mux2/3
  [Vx] -> Mux3/1
  [y] -> Mux2/2
  Mux/1 -> Orientation_dot/1
  [Vy] -> Mux3/2
  Mux1/1 -> Orientation/1
  [x] -> Mux2/1
  Constant2/1 -> Mux/1
  [ax] -> Mux4/1
  Mux4/1 -> Acc/1
  [az] -> Mux4/3
  [Vz] -> Mux3/3
  [ay] -> Mux4/2
  Mux2/1 -> Pose/1
  Mux3/1 -> Vel/1
  2 Wheels Diffrential Mobile Robot/8(Vz) -> [Vz]
  2 Wheels Diffrential Mobile Robot/7(Z) -> [z]
  2 Wheels Diffrential Mobile Robot/4(Y) -> [y]
  2 Wheels Diffrential Mobile Robot/1(X) -> [x]
  2 Wheels Diffrential Mobile Robot/9(az) -> [az]
  2 Wheels Diffrential Mobile Robot/3(ax) -> [ax]
  2 Wheels Diffrential Mobile Robot/10(yaw) -> [yaw]
  2 Wheels Diffrential Mobile Robot/6(ay) -> [ay]
  2 Wheels Diffrential Mobile Robot/5(Vy) -> [Vy]
  2 Wheels Diffrential Mobile Robot/2(Vx) -> [Vx]
  Constant3/1 -> Mux/2
  Constant1/1 -> Mux1/2
  [yaw] -> Mux1/3
  [yaw_dot] -> Mux/3
  2 Wheels Diffrential Mobile Robot/11(yaw_dot) -> [yaw_dot]
  MATLAB Function7/2(Ty_R) -> 2 Wheels Diffrential Mobile Robot/4(Ty)
  MATLAB Function7/1(Tx_R) -> 2 Wheels Diffrential Mobile Robot/3(Tx)
  MATLAB Function7/3(Tz_R) -> 2 Wheels Diffrential Mobile Robot/5(Tz)
  [yaw] -> Delay22/1
  Delay22/1 -> IC/1
  T_L1_MP/1 -> MATLAB Function7/1(T_Global)
  Constant4/1 -> MATLAB Function7/2(roll)
  Constant5/1 -> MATLAB Function7/3(pitch)
  IC/1 -> MATLAB Function7/4(yaw)

== system cable_driven_parallel_robot/Actuators-CableTension-MovingPlatform/2 Wheels Diffrential Mobile Robot1 ==
  TR : Inport
  TL : Inport  Port=2
  T_L2_MP : Inport  Port=3
  2 Wheels Diffrential Mobile Robot : Subsystem
  Constant{,1..5} (6 alike) : Constant  Value=0
  Constant17 : Constant  Value=MR_Jr
  Constant18 : Constant  Value=MR_m
  Constant19 : Constant  Value=MR_r
  Constant20 : Constant  Value=MR_WT
  Delay22 : Delay  DelayLength=1
  IC : InitialCondition  Value=MR_init_Yaw_L2
  MATLAB Function7 : MATLAB Function  TreatAsAtomicUnit=on
  Mux{,1..4} (5 alike) : Mux  Inputs=3
  Pose : Outport
  Vel : Outport  Port=2
  Acc : Outport  Port=3
  Orientation : Outport  Port=4
  Orientation_dot : Outport  Port=5
  wires:
  IC/1 -> MATLAB Function7/4(yaw)
  Constant5/1 -> MATLAB Function7/3(pitch)
  Constant4/1 -> MATLAB Function7/2(roll)
  T_L2_MP/1 -> MATLAB Function7/1(T_Global)
  Delay22/1 -> IC/1
  [yaw] -> Delay22/1
  MATLAB Function7/3(Tz_R) -> 2 Wheels Diffrential Mobile Robot/5(Tz)
  MATLAB Function7/1(Tx_R) -> 2 Wheels Diffrential Mobile Robot/3(Tx)
  MATLAB Function7/2(Ty_R) -> 2 Wheels Diffrential Mobile Robot/4(Ty)
  2 Wheels Diffrential Mobile Robot/11(yaw_dot) -> [yaw_dot]
  [yaw_dot] -> Mux/3
  [yaw] -> Mux1/3
  Constant1/1 -> Mux1/2
  Constant3/1 -> Mux/2
  2 Wheels Diffrential Mobile Robot/2(Vx) -> [Vx]
  2 Wheels Diffrential Mobile Robot/5(Vy) -> [Vy]
  2 Wheels Diffrential Mobile Robot/6(ay) -> [ay]
  2 Wheels Diffrential Mobile Robot/10(yaw) -> [yaw]
  2 Wheels Diffrential Mobile Robot/3(ax) -> [ax]
  2 Wheels Diffrential Mobile Robot/9(az) -> [az]
  2 Wheels Diffrential Mobile Robot/1(X) -> [x]
  2 Wheels Diffrential Mobile Robot/4(Y) -> [y]
  2 Wheels Diffrential Mobile Robot/7(Z) -> [z]
  2 Wheels Diffrential Mobile Robot/8(Vz) -> [Vz]
  Mux3/1 -> Vel/1
  Mux2/1 -> Pose/1
  [ay] -> Mux4/2
  [Vz] -> Mux3/3
  [az] -> Mux4/3
  Mux4/1 -> Acc/1
  [ax] -> Mux4/1
  Constant2/1 -> Mux/1
  [x] -> Mux2/1
  Mux1/1 -> Orientation/1
  [Vy] -> Mux3/2
  Mux/1 -> Orientation_dot/1
  [y] -> Mux2/2
  [Vx] -> Mux3/1
  [z] -> Mux2/3
  Constant/1 -> Mux1/1
  TR/1 -> 2 Wheels Diffrential Mobile Robot/1(TR)
  TL/1 -> 2 Wheels Diffrential Mobile Robot/2(TL)
  Constant20/1 -> 2 Wheels Diffrential Mobile Robot/9(Wheel Track)
  Constant18/1 -> 2 Wheels Diffrential Mobile Robot/7(mass)
  Constant17/1 -> 2 Wheels Diffrential Mobile Robot/6(Jr)
  Constant19/1 -> 2 Wheels Diffrential Mobile Robot/8(r)

== system cable_driven_parallel_robot/Actuators-CableTension-MovingPlatform/2 Wheels Diffrential Mobile Robot2 ==
  TR : Inport
  TL : Inport  Port=2
  T_L3_MP : Inport  Port=3
  2 Wheels Diffrential Mobile Robot : Subsystem
  Constant{,1..5} (6 alike) : Constant  Value=0
  Constant17 : Constant  Value=MR_Jr
  Constant18 : Constant  Value=MR_m
  Constant19 : Constant  Value=MR_r
  Constant20 : Constant  Value=MR_WT
  Delay22 : Delay  DelayLength=1
  IC : InitialCondition  Value=MR_init_Yaw_L3
  MATLAB Function7 : MATLAB Function  TreatAsAtomicUnit=on
  Mux{,1..4} (5 alike) : Mux  Inputs=3
  Pose : Outport
  Vel : Outport  Port=2
  Acc : Outport  Port=3
  Orientation : Outport  Port=4
  Orientation_dot : Outport  Port=5
  wires:
  IC/1 -> MATLAB Function7/4(yaw)
  Constant5/1 -> MATLAB Function7/3(pitch)
  Constant4/1 -> MATLAB Function7/2(roll)
  T_L3_MP/1 -> MATLAB Function7/1(T_Global)
  Delay22/1 -> IC/1
  [yaw] -> Delay22/1
  MATLAB Function7/3(Tz_R) -> 2 Wheels Diffrential Mobile Robot/5(Tz)
  MATLAB Function7/1(Tx_R) -> 2 Wheels Diffrential Mobile Robot/3(Tx)
  MATLAB Function7/2(Ty_R) -> 2 Wheels Diffrential Mobile Robot/4(Ty)
  2 Wheels Diffrential Mobile Robot/11(yaw_dot) -> [yaw_dot]
  [yaw_dot] -> Mux/3
  [yaw] -> Mux1/3
  Constant1/1 -> Mux1/2
  Constant3/1 -> Mux/2
  2 Wheels Diffrential Mobile Robot/2(Vx) -> [Vx]
  2 Wheels Diffrential Mobile Robot/5(Vy) -> [Vy]
  2 Wheels Diffrential Mobile Robot/6(ay) -> [ay]
  2 Wheels Diffrential Mobile Robot/10(yaw) -> [yaw]
  2 Wheels Diffrential Mobile Robot/3(ax) -> [ax]
  2 Wheels Diffrential Mobile Robot/9(az) -> [az]
  2 Wheels Diffrential Mobile Robot/1(X) -> [x]
  2 Wheels Diffrential Mobile Robot/4(Y) -> [y]
  2 Wheels Diffrential Mobile Robot/7(Z) -> [z]
  2 Wheels Diffrential Mobile Robot/8(Vz) -> [Vz]
  Mux3/1 -> Vel/1
  Mux2/1 -> Pose/1
  [ay] -> Mux4/2
  [Vz] -> Mux3/3
  [az] -> Mux4/3
  Mux4/1 -> Acc/1
  [ax] -> Mux4/1
  Constant2/1 -> Mux/1
  [x] -> Mux2/1
  Mux1/1 -> Orientation/1
  [Vy] -> Mux3/2
  Mux/1 -> Orientation_dot/1
  [y] -> Mux2/2
  [Vx] -> Mux3/1
  [z] -> Mux2/3
  Constant/1 -> Mux1/1
  TR/1 -> 2 Wheels Diffrential Mobile Robot/1(TR)
  TL/1 -> 2 Wheels Diffrential Mobile Robot/2(TL)
  Constant20/1 -> 2 Wheels Diffrential Mobile Robot/9(Wheel Track)
  Constant18/1 -> 2 Wheels Diffrential Mobile Robot/7(mass)
  Constant17/1 -> 2 Wheels Diffrential Mobile Robot/6(Jr)
  Constant19/1 -> 2 Wheels Diffrential Mobile Robot/8(r)

== system cable_driven_parallel_robot/Actuators-CableTension-MovingPlatform/2 Wheels Diffrential Mobile Robot3 ==
  TR : Inport
  TL : Inport  Port=2
  T_L4_MP : Inport  Port=3
  2 Wheels Diffrential Mobile Robot : Subsystem
  Constant{,1..5} (6 alike) : Constant  Value=0
  Constant17 : Constant  Value=MR_Jr
  Constant18 : Constant  Value=MR_m
  Constant19 : Constant  Value=MR_r
  Constant20 : Constant  Value=MR_WT
  Delay22 : Delay  DelayLength=1
  IC : InitialCondition  Value=MR_init_Yaw_L4
  MATLAB Function7 : MATLAB Function  TreatAsAtomicUnit=on
  Mux{,1..4} (5 alike) : Mux  Inputs=3
  Pose : Outport
  Vel : Outport  Port=2
  Acc : Outport  Port=3
  Orientation : Outport  Port=4
  Orientation_dot : Outport  Port=5
  wires:
  IC/1 -> MATLAB Function7/4(yaw)
  Constant5/1 -> MATLAB Function7/3(pitch)
  Constant4/1 -> MATLAB Function7/2(roll)
  T_L4_MP/1 -> MATLAB Function7/1(T_Global)
  Delay22/1 -> IC/1
  [yaw] -> Delay22/1
  MATLAB Function7/3(Tz_R) -> 2 Wheels Diffrential Mobile Robot/5(Tz)
  MATLAB Function7/1(Tx_R) -> 2 Wheels Diffrential Mobile Robot/3(Tx)
  MATLAB Function7/2(Ty_R) -> 2 Wheels Diffrential Mobile Robot/4(Ty)
  2 Wheels Diffrential Mobile Robot/11(yaw_dot) -> [yaw_dot]
  [yaw_dot] -> Mux/3
  [yaw] -> Mux1/3
  Constant1/1 -> Mux1/2
  Constant3/1 -> Mux/2
  2 Wheels Diffrential Mobile Robot/2(Vx) -> [Vx]
  2 Wheels Diffrential Mobile Robot/5(Vy) -> [Vy]
  2 Wheels Diffrential Mobile Robot/6(ay) -> [ay]
  2 Wheels Diffrential Mobile Robot/10(yaw) -> [yaw]
  2 Wheels Diffrential Mobile Robot/3(ax) -> [ax]
  2 Wheels Diffrential Mobile Robot/9(az) -> [az]
  2 Wheels Diffrential Mobile Robot/1(X) -> [x]
  2 Wheels Diffrential Mobile Robot/4(Y) -> [y]
  2 Wheels Diffrential Mobile Robot/7(Z) -> [z]
  2 Wheels Diffrential Mobile Robot/8(Vz) -> [Vz]
  Mux3/1 -> Vel/1
  Mux2/1 -> Pose/1
  [ay] -> Mux4/2
  [Vz] -> Mux3/3
  [az] -> Mux4/3
  Mux4/1 -> Acc/1
  [ax] -> Mux4/1
  Constant2/1 -> Mux/1
  [x] -> Mux2/1
  Mux1/1 -> Orientation/1
  [Vy] -> Mux3/2
  Mux/1 -> Orientation_dot/1
  [y] -> Mux2/2
  [Vx] -> Mux3/1
  [z] -> Mux2/3
  Constant/1 -> Mux1/1
  TR/1 -> 2 Wheels Diffrential Mobile Robot/1(TR)
  TL/1 -> 2 Wheels Diffrential Mobile Robot/2(TL)
  Constant20/1 -> 2 Wheels Diffrential Mobile Robot/9(Wheel Track)
  Constant18/1 -> 2 Wheels Diffrential Mobile Robot/7(mass)
  Constant17/1 -> 2 Wheels Diffrential Mobile Robot/6(Jr)
  Constant19/1 -> 2 Wheels Diffrential Mobile Robot/8(r)
